simulink model "MCS_CLA03STATEFEEDBACK"  (R2023b)
settings: Solver=VariableStepAuto  StartTime=0.0  StopTime=10.0  RelTol=1e-3
values from neighbouring files (symbols this model uses):
  A = [-1 0 0 0; 1 0 -1 0; 0 -1 1 0; 0 -1 0 0; 0 1 0 -1; -1 0 0 1]    [PSA_ex1.m]
  K = 1/mag    [MCS_Ex06.m]    (also in MCS_Ex06_rootlocus_code.m = 10)
undefined symbols (not defined in the file or in its folder): B, C
settings Model: Creator=lalit  LastModifiedBy=lalit

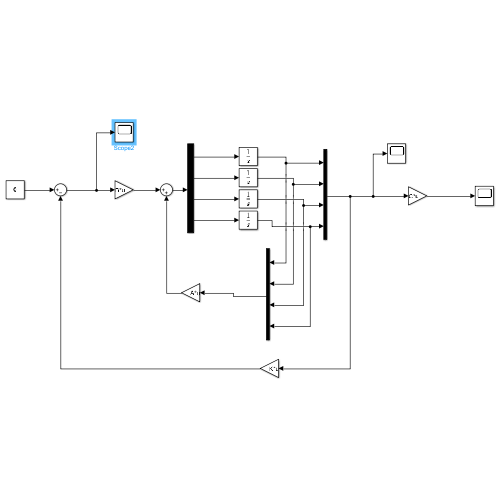
[thumbnail: Simulink's stored preview of the top-level diagram]
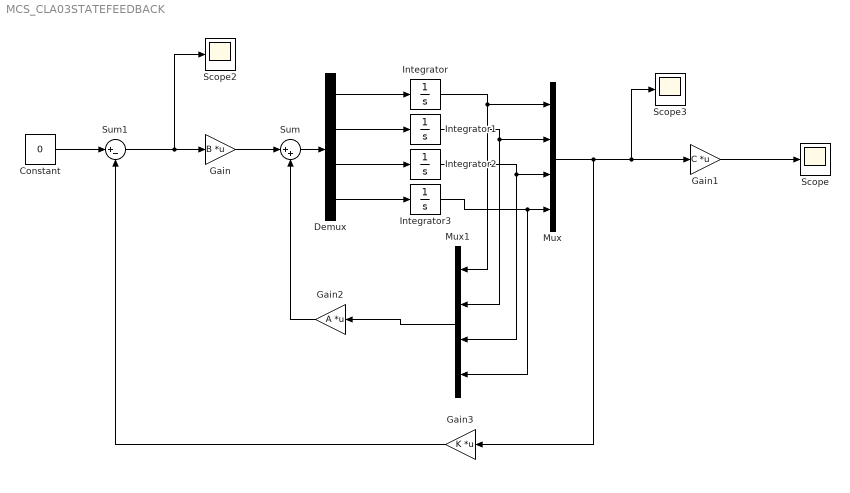
== system MCS_CLA03STATEFEEDBACK ==
  Constant : Constant  Value=0
  Demux : Demux
  Gain : Gain  Gain=B  Multiplication=Matrix(K*u)
  Gain1 : Gain  Gain=C  Multiplication=Matrix(K*u)
  Gain2 : Gain  Gain=A  Multiplication=Matrix(K*u)
  Gain3 : Gain  Gain=K  Multiplication=Matrix(K*u)
  Integrator : Integrator
  Integrator1 : Integrator  InitialCondition=0.01
  Integrator2 : Integrator
  Integrator3 : Integrator
  Mux : Mux
  Mux1 : Mux
  Scope : Scope
  Scope2 : Scope
  Scope3 : Scope
  Sum : Sum  Inputs=|++
  Sum1 : Sum  Inputs=|+-
  wires:
  Integrator/1 -> Mux/1, Mux1/1
  Integrator1/1 -> Mux/2, Mux1/2
  Integrator2/1 -> Mux1/3, Mux/3
  Integrator3/1 -> Mux1/4, Mux/4
  Mux/1 -> Gain3/1, Scope3/1, Gain1/1
  Gain/1 -> Sum/1
  Sum1/1 -> Scope2/1, Gain/1
  Mux1/1 -> Gain2/1
  Gain2/1 -> Sum/2
  Gain3/1 -> Sum1/2
  Constant/1 -> Sum1/1
  Gain1/1 -> Scope/1
  Sum/1 -> Demux/1
  Demux/1 -> Integrator/1
  Demux/2 -> Integrator1/1
  Demux/3 -> Integrator2/1
  Demux/4 -> Integrator3/1
